simulink model "FSI_2DOF_sim"  (R2018b)
settings: Solver=VariableStepAuto  StartTime=0.0  StopTime=1  FixedStep=time_step  RelTol=0.1*dt  EnableMultiTasking=on
undefined symbols (not defined in the file): b1, b2, dt, dx10, dx20, f1_a, f1_fi, f1_freq, f2_a, f2_fi, f2_freq, joint_control, k1, k2, m1, m2, pb_1, pb_2, step_time_1, step_time_2, step_width_1, step_width_2, x10, x20
settings Model: Creator=Phil  LastModifiedBy=FilipKsica
settings DataIOCC: LimitDataPoints=on  SaveFormat=Array
settings OptimizationCC: LifeSpan=inf
settings DebuggingCC: UnderspecifiedInitializationDetection=Classic  MergeDetectMultiDrivingBlocksExec=none  SolverPrmCheckMsg=warning  AllowSymbolicDim=off  StateNameClashWarn=warning  SFUnexpectedBacktrackingDiag=warning  SFNoUnconditionalDefaultTransitionDiag=warning  SFExecutionAtInitializationDiag=none
settings HardwareCC: ProdBitPerPointer=32  ProdBitPerSizeT=32  ProdBitPerPtrDiffT=32  ProdLargestAtomicFloat=None  ProdIntDivRoundTo=Undefined  ProdEndianess=Unspecified  ProdWordSize=32  ProdHWDeviceType=32-bit Generic
settings ModelReferenceCC: PropagateSignalLabelsOutOfModel=off
settings SFSimCC: SimUseLocalCustomCode=off
settings RTWCC: RTWUseLocalCustomCode=off
settings CodeAppCC: StateflowObjectComments=on
settings GRTTargetCC: TargetLangStandard=C89/C90 (ANSI)  GeneratePreprocessorConditionals=Disable all
settings ConfigComp: CovMetricSettings=dw  CovHtmlReporting=on  CovSaveCumulativeToWorkspaceVar=on  CovSaveSingleToWorkspaceVar=on  CovExternalEMLEnable=off

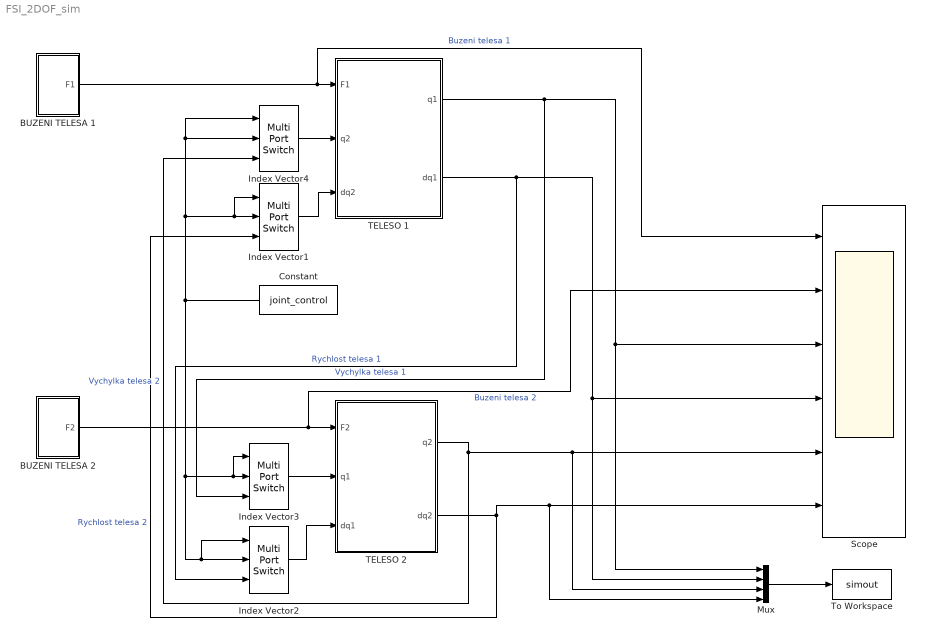
== system FSI_2DOF_sim ==
  BUZENI TELESA 1 : Subsystem
  BUZENI TELESA 2 : Subsystem
  Constant : Constant  Value=joint_control
  Index Vector{1..4} (4 alike) : MultiPortSwitch  DataPortOrder=Zero-based contiguous  Inputs=2  zeroidx=on
  Mux : Mux
  Scope : Scope  NumInputPorts=6
  TELESO 1 : Subsystem
  TELESO 2 : Subsystem
  To Workspace : ToWorkspace  VariableName=simout  SampleTime=-1
  wires:
  Index Vector3/1 -> TELESO 2/2(q1)
  Index Vector2/1 -> TELESO 2/3(dq1)
  TELESO 2/1(q2) -> Index Vector4/3, Scope/5, Mux/3  "Vychylka telesa 2"
  Mux/1 -> To Workspace/1
  BUZENI TELESA 2/1(F2) -> Scope/2, TELESO 2/1(F2)  "Buzeni telesa 2"
  BUZENI TELESA 1/1(F1) -> Scope/1, TELESO 1/1(F1)  "Buzeni telesa 1"
  TELESO 1/2(dq1) -> Mux/2, Scope/4, Index Vector2/3  "Rychlost telesa 1"
  TELESO 1/1(q1) -> Scope/3, Mux/1, Index Vector3/3  "Vychylka telesa 1"
  Index Vector1/1 -> TELESO 1/3(dq2)
  Index Vector4/1 -> TELESO 1/2(q2)
  Constant/1 -> Index Vector4/1, Index Vector4/2, Index Vector1/2, Index Vector1/1, Index Vector2/2, Index Vector2/1, Index Vector3/2, Index Vector3/1
  TELESO 2/2(dq2) -> Scope/6, Mux/4, Index Vector1/3  "Rychlost telesa 2"

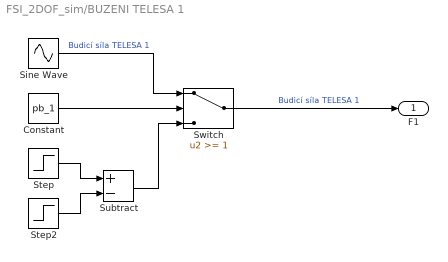
== system FSI_2DOF_sim/BUZENI TELESA 1 ==
  Constant : Constant  Value=pb_1
  Sine Wave : Sin  Amplitude=f1_a  Frequency=f1_freq  Phase=f1_fi  SampleTime=dt
  Step : Step  Time=step_time_1  After=f1_a  SampleTime=0
  Step2 : Step  Time=step_time_1+step_width_1  After=f1_a  SampleTime=0
  Subtract : Sum  Inputs=+-
  Switch : Switch  Threshold=1
  F1 : Outport
  wires:
  Switch/1 -> F1/1  "Budicí síla TELESA 1"
  Sine Wave/1 -> Switch/1  "Budicí síla TELESA 1"
  Constant/1 -> Switch/2
  Subtract/1 -> Switch/3
  Step/1 -> Subtract/1
  Step2/1 -> Subtract/2

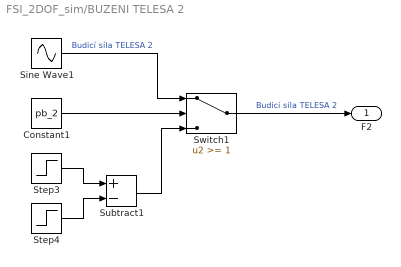
== system FSI_2DOF_sim/BUZENI TELESA 2 ==
  Constant1 : Constant  Value=pb_2
  Sine Wave1 : Sin  Amplitude=f2_a  Frequency=f2_freq  Phase=f2_fi  SampleTime=dt
  Step3 : Step  Time=step_time_2  After=f2_a  SampleTime=0
  Step4 : Step  Time=step_time_2+step_width_2  After=f2_a  SampleTime=0
  Subtract1 : Sum  Inputs=+-
  Switch1 : Switch  Threshold=1
  F2 : Outport
  wires:
  Switch1/1 -> F2/1  "Budicí síla TELESA 2"
  Constant1/1 -> Switch1/2
  Sine Wave1/1 -> Switch1/1  "Budicí síla TELESA 2"
  Subtract1/1 -> Switch1/3
  Step3/1 -> Subtract1/1
  Step4/1 -> Subtract1/2

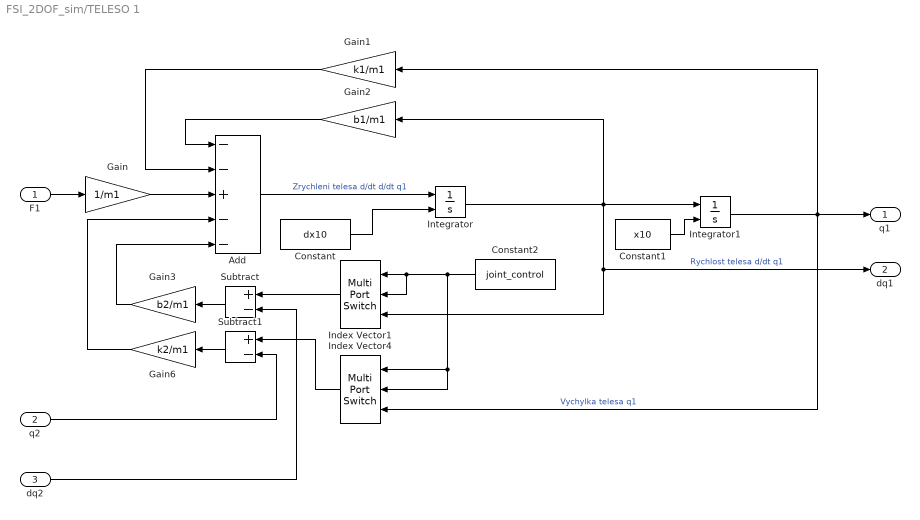
== system FSI_2DOF_sim/TELESO 1 ==
  F1 : Inport
  q2 : Inport  Port=2
  dq2 : Inport  Port=3
  Add : Sum  Inputs=--+--
  Constant : Constant  Value=dx10
  Constant1 : Constant  Value=x10
  Constant2 : Constant  Value=joint_control
  Gain : Gain  Gain=1/m1
  Gain1 : Gain  Gain=k1/m1
  Gain2 : Gain  Gain=b1/m1
  Gain3 : Gain  Gain=b2/m1
  Gain6 : Gain  Gain=k2/m1
  Index Vector1 : MultiPortSwitch  DataPortOrder=Zero-based contiguous  Inputs=2  zeroidx=on
  Index Vector4 : MultiPortSwitch  DataPortOrder=Zero-based contiguous  Inputs=2  zeroidx=on
  Integrator : Integrator  InitialConditionSource=external
  Integrator1 : Integrator  InitialConditionSource=external
  Subtract : Sum  Inputs=+-
  Subtract1 : Sum  Inputs=+-
  q1 : Outport
  dq1 : Outport  Port=2
  wires:
  Subtract/1 -> Gain3/1
  Subtract1/1 -> Gain6/1
  Gain1/1 -> Add/2
  Gain2/1 -> Add/1
  Add/1 -> Integrator/1  "Zrychleni telesa d/dt d/dt q1"
  Integrator1/1 -> Index Vector4/3, q1/1, Gain1/1  "Vychylka telesa q1"
  Integrator/1 -> Gain2/1, Integrator1/1, dq1/1, Index Vector1/3  "Rychlost telesa d/dt q1"
  Gain3/1 -> Add/5
  Gain6/1 -> Add/4
  Gain/1 -> Add/3
  F1/1 -> Gain/1
  dq2/1 -> Subtract/2
  q2/1 -> Subtract1/2
  Constant/1 -> Integrator/2
  Constant1/1 -> Integrator1/2
  Constant2/1 -> Index Vector4/2, Index Vector4/1, Index Vector1/2, Index Vector1/1
  Index Vector1/1 -> Subtract/1
  Index Vector4/1 -> Subtract1/1

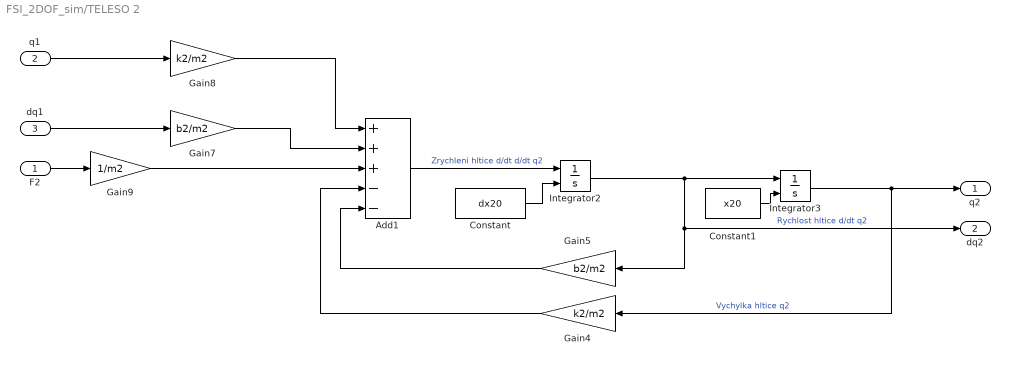
== system FSI_2DOF_sim/TELESO 2 ==
  F2 : Inport
  q1 : Inport  Port=2
  dq1 : Inport  Port=3
  Add1 : Sum  Inputs=+++--
  Constant : Constant  Value=dx20
  Constant1 : Constant  Value=x20
  Gain4 : Gain  Gain=k2/m2
  Gain5 : Gain  Gain=b2/m2
  Gain7 : Gain  Gain=b2/m2
  Gain8 : Gain  Gain=k2/m2
  Gain9 : Gain  Gain=1/m2
  Integrator2 : Integrator  InitialConditionSource=external
  Integrator3 : Integrator  InitialConditionSource=external
  q2 : Outport
  dq2 : Outport  Port=2
  wires:
  Integrator2/1 -> Integrator3/1, dq2/1, Gain5/1  "Rychlost hltice d/dt q2"
  Integrator3/1 -> Gain4/1, q2/1  "Vychylka hltice q2"
  Add1/1 -> Integrator2/1  "Zrychleni hltice d/dt d/dt q2"
  Gain5/1 -> Add1/5
  Gain4/1 -> Add1/4
  Gain9/1 -> Add1/3
  Gain8/1 -> Add1/1
  Gain7/1 -> Add1/2
  F2/1 -> Gain9/1
  q1/1 -> Gain8/1
  dq1/1 -> Gain7/1
  Constant1/1 -> Integrator3/2
  Constant/1 -> Integrator2/2
